simulink model "Intro_PID_Demo"  (R2025b)
settings: Solver=ode45  StartTime=0.0  StopTime=15  MaxStep=0.001  RelTol=1e-6  AbsTol=1e-8
InitFcn:
  | evalin(get_param(bdroot,'ModelWorkspace'),'assert(m>0 && g>0 && a>0 && I>0, ''Physical parameters must be positive.''); assert(F_max>m*g && phi_max>0, ''Limits must allow hover and gimbal movement.''); assert(theta_max>0 && theta_max<=pi/6, ''Use a small positive tilt-command limit.''); assert(numel(X0)==6 && numel(Xref)==6, ''X0 and Xref need six states.''); assert(all(Xref([2 4 5 6])==0), ''Use stationary upright position references.''); assert(all([Kp_x Kd_x Kp_y Kd_y Kp_theta Kd_theta]>0), ''P and D gains must be positive.''); assert(all([Ki_x Ki_y Ki_theta]>=0), ''Integral gains must be nonnegative.'');');
model workspace (MAT data in the model file):
  F_max = 20
  I = 1
  Kd_theta = 1.10091743119
  Kd_x = 1
  Kd_y = 3
  Ki_theta = 0
  Ki_x = 0
  Ki_y = 0
  Kp_theta = 3.66972477064
  Kp_x = 0.25
  Kp_y = 1
  Ts_noise = 0.01
  X0 = [2; 0; 0; 0; 0.03; 0]
  Xref = [3; 0; 30; 0; 0; 0]
  a = 1
  g = 9.81
  m = 1
  phi_max = 0.17
  sigma = [0.03; 0.06; 0.03; 0.06; 0.006; 0.009]
  theta_max = 0.17
libraries: slpidlib x3, simulink x1
settings Model: Creator=cmax0  LastModifiedBy=cmax0

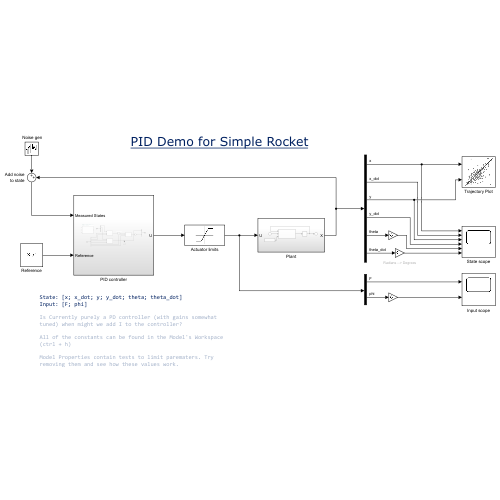
[thumbnail: Simulink's stored preview of the top-level diagram]
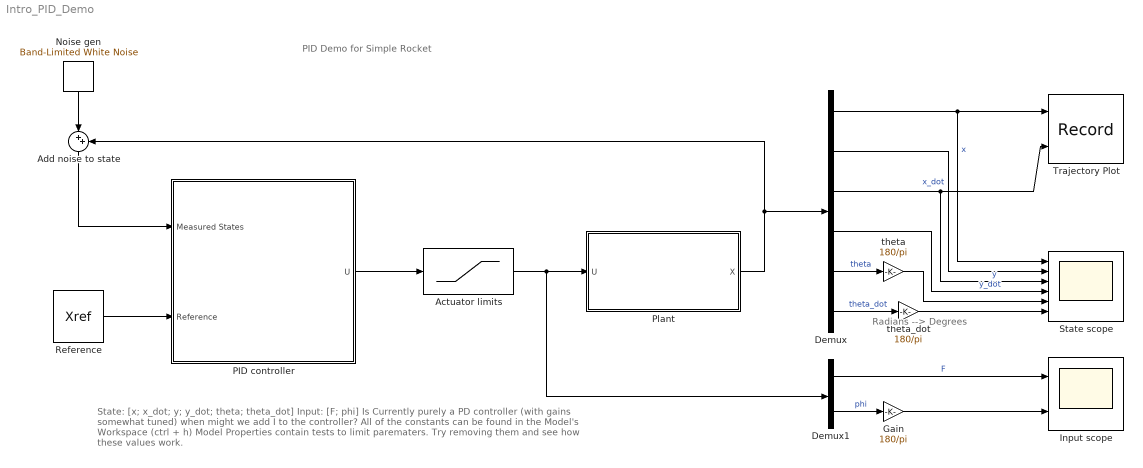
== system Intro_PID_Demo ==
  note: PID Demo for Simple Rocket
  note: State: [x; x_dot; y; y_dot; theta; theta_dot]
      | Input: [F; phi]
      |
      | Is Currently purely a PD controller (with gains somewhat tuned) when might we add I to the controller?
      |
      | All of the constants can be found in the Model's Workspace (ctrl + h)
      |
      | Model Properties contain tests to limit parematers. Try removing them and see how these values work.
  note: Radians --> Degrees
  " Noise gen" : simulink/Sources/Band-Limited White Noise  Cov=sigma.^2 * Ts_noise  Ts=Ts_noise  seed=[11;22;33;44;55;66]
  Actuator limits : Saturate  UpperLimit=[F_max;phi_max]  LowerLimit=[0;-phi_max]
  Add noise to state : Sum  Inputs=|++
  Demux : Demux  Outputs=6
  Demux1 : Demux  Outputs=2
  Gain : Gain  Gain=180/pi
  Input scope : Scope  NumInputPorts=2
      settings: ActiveDisplayYMinimum=-9.207816529611673  ActiveDisplayYMaximum=33.207701324124656
  PID controller : Subsystem
  Plant : Subsystem
  Reference : Constant  Value=Xref
  State scope : Scope  NumInputPorts=6
      settings: ActiveDisplayYMinimum=-27.6164299238122  ActiveDisplayYMaximum=55.714795015888747
  Trajectory Plot : Record  NumPorts=2.0  FileSettingsInternal="{\"entries\":[{\"content\":{\"excelSettings\":{\"content\":{},\"type\":\"Streamout.ExcelSettings\"},\"parquetSettings\":{\"content\":{},\"type\":\"Streamout.ParquetSettings\"}},\"type\":\"Streamout.FileSettingStorage\",\"uuid\":\"\"}],\"packageUris\":[\"http:\\/\\/schema.mathworks.com\\/mf0\\/streamout_blocks\\/R2020a\"],\"version\":\"1.0\"}"  FrameSettings=[0, 0]  Layout=[1 1]  SignalsInternal="{\"entries\":[{\"content\":{\"signals\":[{\"content\":{\"blockPath\":[],\"dimensions\":[1,1],\"domain\":\"\",\"lineColor\":\"#a2142f\",\"plots\":[ 1 ],\"port\":1,\"sid\":[\"\"],\"signalID\":1,\"signalName\":\"x\"},\"type\":\"RecordBlkView.Signal\",\"uuid\":\"\"},{\"content\":{\"blockPath\":[],\"dimensions\":[1,1],\"domain\":\"\",\"lineColor\":\"#139fff\",\"plots\":[ 1 ],\"port\":2,\"sid\":[\"\"],\"signalID\":2,\"signalName\":\"y\"},\"type\":\"RecordBlkView.Signal\",\"uuid\":\"\"}]},\"type\":\"RecordBlkView.InputSignals\",\"uuid\":\"\"}],\"packageUris\":[\"http:\\/\\/schema.mathworks.com\\/mf0\\/streamout_blocks\\/R2020a\"],\"version\":\"1.0\"}"  VisualizationBindings="{\"xyplotplugin\":{\"info\":[{\"series\":[{\"bindingParametersList\":[{\"parameter\":\"X-Axis\",\"signalID\":1,\"signalName\":\"x\"},{\"parameter\":\"Y-Axis\",\"signalID\":2,\"signalName\":\"y\"}],\"seriesID\":0}],\"subplotID\":1}]}}"  CompatibilityTag=XY
  theta : Gain  Gain=180/pi
  theta_dot : Gain  Gain=180/pi
  wires:
  Plant/1(X) -> Add noise to state/2, Demux/1
  Actuator limits/1 -> Plant/1(U), Demux1/1
  " Noise gen"/1 -> Add noise to state/1
  Demux/1 -> Trajectory Plot/1, State scope/1  "x"
  Demux/2 -> State scope/2  "x_dot"
  Demux/3 -> State scope/3, Trajectory Plot/2  "y"
  Demux/5 -> theta/1  "theta"
  Demux/6 -> theta_dot/1  "theta_dot"
  Demux/4 -> State scope/4  "y_dot"
  Demux1/1 -> Input scope/1  "F"
  Demux1/2 -> Gain/1  "phi"
  Reference/1 -> PID controller/2(Reference)
  Add noise to state/1 -> PID controller/1(Measured States)
  PID controller/1(U) -> Actuator limits/1
  Gain/1 -> Input scope/2
  theta_dot/1 -> State scope/6
  theta/1 -> State scope/5

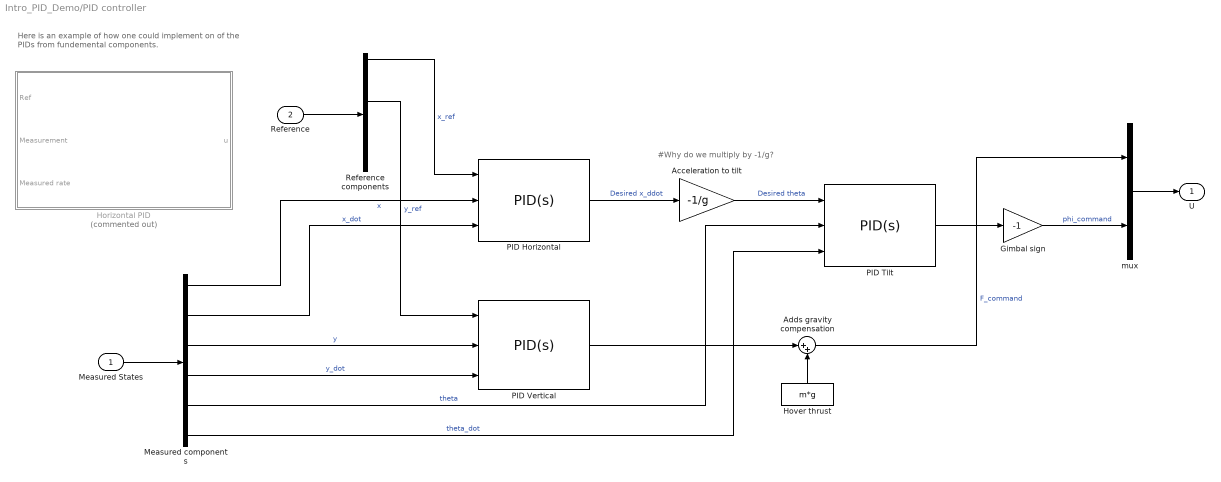
== system Intro_PID_Demo/PID controller ==
  note: Here is an example of how one could implement on of the PIDs from fundemental components.
  note: #Why do we multiply by -1/g?
  Measured States : Inport
  Reference : Inport  Port=2
  Acceleration to tilt : Gain  Gain=-1/g
  Adds gravity compensation : Sum  Inputs=|++
  Gimbal sign : Gain  Gain=-1
  Horizontal PID : Subsystem  Commented=on
  Hover thrust : Constant  Value=m*g
  Measured components : Demux  Outputs=6
  PID Horizontal : slpidlib/PID Controller (2DOF)  Controller=PID  Form=Parallel  TimeDomain=Continuous-time  UseExternalTs=off  SampleTime=-1  IntegratorMethod=Forward Euler  FilterMethod=Forward Euler  ControllerParametersSource=internal  P=Kp_x  I=Ki_x  UseKiTs=off  D=Kd_x  UseExternalDerivativeSource=on  N=100  UseFilter=on  b=1  c=0  TunerSelectOption=Transfer Function Based (PID Tuner App)  InitialConditionSource=internal  InitialConditionForIntegrator=0  InitialConditionForFilter=0  DifferentiatorICPrevScaledInput=0  ExternalReset=none  TrackingMode=off  Kt=1  LimitOutput=on  SatLimitsSource=internal  UpperSaturationLimit=theta_max*g  LowerSaturationLimit=-theta_max*g  LinearizeAsGain=on  AntiWindupMode=clamping  Kb=1  LimitIntegrator=off  UpperIntegratorSaturationLimit=inf  LowerIntegratorSaturationLimit=-inf  POutMin=[]  POutMax=[]  IOutMin=[]  IOutMax=[]  DOutMin=[]  DOutMax=[]  NOutMin=[]  NOutMax=[]  bOutMin=[]  bOutMax=[]  cOutMin=[]  cOutMax=[]  SumOutMin=[]  SumOutMax=[]  SaturationOutMin=[]  SaturationOutMax=[]  PParamMin=[]  PParamMax=[]  IParamMin=[]  IParamMax=[]  DParamMin=[]  DParamMax=[]  NParamMin=[]  NParamMax=[]  bParamMin=[]  bParamMax=[]  cParamMin=[]  cParamMax=[]  KbParamMin=[]  KbParamMax=[]  KtParamMin=[]  KtParamMax=[]  KbOutMin=[]  KbOutMax=[]  KtOutMin=[]  KtOutMax=[]  IntegratorOutMin=[]  IntegratorOutMax=[]  FilterOutMin=[]  FilterOutMax=[]  SumI1OutMin=[]  SumI1OutMax=[]  SumI2OutMin=[]  SumI2OutMax=[]  SumI3OutMin=[]  SumI3OutMax=[]  SumI4OutMin=[]  SumI4OutMax=[]  SumDOutMin=[]  SumDOutMax=[]  Sum1OutMin=[]  Sum1OutMax=[]  Sum2OutMin=[]  Sum2OutMax=[]  Sum3OutMin=[]  Sum3OutMax=[]  DifferentiatorOutMin=[]  DifferentiatorOutMax=[]  FilterDiffOutCoefMin=[]  FilterDiffOutCoefMax=[]  ReciprocalOutMin=[]  ReciprocalOutMax=[]  SumDenOutMin=[]  SumDenOutMax=[]  SumNumOutMin=[]  SumNumOutMax=[]  DivideOutMin=[]  DivideOutMax=[]  UdiffTsProdOutMin=[]  UdiffTsProdOutMax=[]  NTsProdOutMin=[]  NTsProdOutMax=[]  UintegralTsProdOutMin=[]  UintegralTsProdOutMax=[]  UngainTsProdOutMin=[]  UngainTsProdOutMax=[]  ClampingZeroOutDataTypeStr=Inherit: Inherit via back propagation  ClampingZeroOutMin=[]  ClampingZeroOutMax=[]  FilterDenConstantOutDataTypeStr=Inherit: Inherit via back propagation  FilterDenConstantOutMin=[]  FilterDenConstantOutMax=[]  PCopyOutDataTypeStr=Inherit: Inherit via back propagation  PCopyOutMin=[]  PCopyOutMax=[]  NCopyOutDataTypeStr=Inherit: Inherit via back propagation  NCopyOutMin=[]  NCopyOutMax=[]  IntegratorContinuousStateAttributes=''  IntegratorStateMustResolveToSignalObject=off  IntegratorRTWStateStorageClass=Auto  FilterContinuousStateAttributes=''  FilterStateMustResolveToSignalObject=off  FilterRTWStateStorageClass=Auto  ParallelPVariant=InternalParameters  IdealPVariant=Disabled  IVariant=InternalParameters  DVariant=InternalParameters  bVariant=InternalParameters  cVariant=Disabled  IntegratorVariant=Continuous  SatVariant=Enabled  AWVariant=ContClampingParallel  PCopyVariant=Disabled  TRVariant=Disabled  FdbkBlocksVariant=Forward  IdealPFdbkVariant=Disabled  SatFdbkVariant=Disabled  DerivativeFilterVariant=ContFilterOnly  NVariant=InternalParameters  NCopyVariant=Disabled  FilterICVariant=InternalICsFilter  IntegratorICVariant=InternalICs  ExternalResetVariant=Disabled  TRSumVariant=Passthrough  SumFdbkVariant=Disabled  SumVariant=Sum_PID  TsampFilterVariant=InternalTs  TsampNgainVariant=Passthrough  TsampIntegralVariant=Disabled_SignalSpec  ExternalSaturationOutDataTypeStr=Inherit: Same as second input  DerivativeSourceVariant=ExternalYdot  PreIntVariant=InternalPreInt
  PID Tilt : slpidlib/PID Controller (2DOF)  Controller=PID  Form=Parallel  TimeDomain=Continuous-time  UseExternalTs=off  SampleTime=-1  IntegratorMethod=Forward Euler  FilterMethod=Forward Euler  ControllerParametersSource=internal  P=Kp_theta  I=Ki_theta  UseKiTs=off  D=Kd_theta  UseExternalDerivativeSource=on  N=100  UseFilter=on  b=1  c=0  TunerSelectOption=Transfer Function Based (PID Tuner App)  InitialConditionSource=internal  InitialConditionForIntegrator=0  InitialConditionForFilter=0  DifferentiatorICPrevScaledInput=0  ExternalReset=none  TrackingMode=off  Kt=1  LimitOutput=on  SatLimitsSource=internal  UpperSaturationLimit=phi_max  LowerSaturationLimit=-phi_max  LinearizeAsGain=on  AntiWindupMode=clamping  Kb=1  LimitIntegrator=off  UpperIntegratorSaturationLimit=inf  LowerIntegratorSaturationLimit=-inf  POutMin=[]  POutMax=[]  IOutMin=[]  IOutMax=[]  DOutMin=[]  DOutMax=[]  NOutMin=[]  NOutMax=[]  bOutMin=[]  bOutMax=[]  cOutMin=[]  cOutMax=[]  SumOutMin=[]  SumOutMax=[]  SaturationOutMin=[]  SaturationOutMax=[]  PParamMin=[]  PParamMax=[]  IParamMin=[]  IParamMax=[]  DParamMin=[]  DParamMax=[]  NParamMin=[]  NParamMax=[]  bParamMin=[]  bParamMax=[]  cParamMin=[]  cParamMax=[]  KbParamMin=[]  KbParamMax=[]  KtParamMin=[]  KtParamMax=[]  KbOutMin=[]  KbOutMax=[]  KtOutMin=[]  KtOutMax=[]  IntegratorOutMin=[]  IntegratorOutMax=[]  FilterOutMin=[]  FilterOutMax=[]  SumI1OutMin=[]  SumI1OutMax=[]  SumI2OutMin=[]  SumI2OutMax=[]  SumI3OutMin=[]  SumI3OutMax=[]  SumI4OutMin=[]  SumI4OutMax=[]  SumDOutMin=[]  SumDOutMax=[]  Sum1OutMin=[]  Sum1OutMax=[]  Sum2OutMin=[]  Sum2OutMax=[]  Sum3OutMin=[]  Sum3OutMax=[]  DifferentiatorOutMin=[]  DifferentiatorOutMax=[]  FilterDiffOutCoefMin=[]  FilterDiffOutCoefMax=[]  ReciprocalOutMin=[]  ReciprocalOutMax=[]  SumDenOutMin=[]  SumDenOutMax=[]  SumNumOutMin=[]  SumNumOutMax=[]  DivideOutMin=[]  DivideOutMax=[]  UdiffTsProdOutMin=[]  UdiffTsProdOutMax=[]  NTsProdOutMin=[]  NTsProdOutMax=[]  UintegralTsProdOutMin=[]  UintegralTsProdOutMax=[]  UngainTsProdOutMin=[]  UngainTsProdOutMax=[]  ClampingZeroOutDataTypeStr=Inherit: Inherit via back propagation  ClampingZeroOutMin=[]  ClampingZeroOutMax=[]  FilterDenConstantOutDataTypeStr=Inherit: Inherit via back propagation  FilterDenConstantOutMin=[]  FilterDenConstantOutMax=[]  PCopyOutDataTypeStr=Inherit: Inherit via back propagation  PCopyOutMin=[]  PCopyOutMax=[]  NCopyOutDataTypeStr=Inherit: Inherit via back propagation  NCopyOutMin=[]  NCopyOutMax=[]  IntegratorContinuousStateAttributes=''  IntegratorStateMustResolveToSignalObject=off  IntegratorRTWStateStorageClass=Auto  FilterContinuousStateAttributes=''  FilterStateMustResolveToSignalObject=off  FilterRTWStateStorageClass=Auto  ParallelPVariant=InternalParameters  IdealPVariant=Disabled  IVariant=InternalParameters  DVariant=InternalParameters  bVariant=InternalParameters  cVariant=Disabled  IntegratorVariant=Continuous  SatVariant=Enabled  AWVariant=ContClampingParallel  PCopyVariant=Disabled  TRVariant=Disabled  FdbkBlocksVariant=Forward  IdealPFdbkVariant=Disabled  SatFdbkVariant=Disabled  DerivativeFilterVariant=ContFilterOnly  NVariant=InternalParameters  NCopyVariant=Disabled  FilterICVariant=InternalICsFilter  IntegratorICVariant=InternalICs  ExternalResetVariant=Disabled  TRSumVariant=Passthrough  SumFdbkVariant=Disabled  SumVariant=Sum_PID  TsampFilterVariant=InternalTs  TsampNgainVariant=Passthrough  TsampIntegralVariant=Disabled_SignalSpec  ExternalSaturationOutDataTypeStr=Inherit: Same as second input  DerivativeSourceVariant=ExternalYdot  PreIntVariant=InternalPreInt
  PID Vertical : slpidlib/PID Controller (2DOF)  Controller=PID  Form=Parallel  TimeDomain=Continuous-time  UseExternalTs=off  SampleTime=-1  IntegratorMethod=Forward Euler  FilterMethod=Forward Euler  ControllerParametersSource=internal  P=Kp_y  I=Ki_y  UseKiTs=off  D=Kd_y  UseExternalDerivativeSource=on  N=100  UseFilter=on  b=1  c=0  TunerSelectOption=Transfer Function Based (PID Tuner App)  InitialConditionSource=internal  InitialConditionForIntegrator=0  InitialConditionForFilter=0  DifferentiatorICPrevScaledInput=0  ExternalReset=none  TrackingMode=off  Kt=1  LimitOutput=on  SatLimitsSource=internal  UpperSaturationLimit=F_max-m*g  LowerSaturationLimit=-m*g  LinearizeAsGain=on  AntiWindupMode=clamping  Kb=1  LimitIntegrator=off  UpperIntegratorSaturationLimit=inf  LowerIntegratorSaturationLimit=-inf  POutMin=[]  POutMax=[]  IOutMin=[]  IOutMax=[]  DOutMin=[]  DOutMax=[]  NOutMin=[]  NOutMax=[]  bOutMin=[]  bOutMax=[]  cOutMin=[]  cOutMax=[]  SumOutMin=[]  SumOutMax=[]  SaturationOutMin=[]  SaturationOutMax=[]  PParamMin=[]  PParamMax=[]  IParamMin=[]  IParamMax=[]  DParamMin=[]  DParamMax=[]  NParamMin=[]  NParamMax=[]  bParamMin=[]  bParamMax=[]  cParamMin=[]  cParamMax=[]  KbParamMin=[]  KbParamMax=[]  KtParamMin=[]  KtParamMax=[]  KbOutMin=[]  KbOutMax=[]  KtOutMin=[]  KtOutMax=[]  IntegratorOutMin=[]  IntegratorOutMax=[]  FilterOutMin=[]  FilterOutMax=[]  SumI1OutMin=[]  SumI1OutMax=[]  SumI2OutMin=[]  SumI2OutMax=[]  SumI3OutMin=[]  SumI3OutMax=[]  SumI4OutMin=[]  SumI4OutMax=[]  SumDOutMin=[]  SumDOutMax=[]  Sum1OutMin=[]  Sum1OutMax=[]  Sum2OutMin=[]  Sum2OutMax=[]  Sum3OutMin=[]  Sum3OutMax=[]  DifferentiatorOutMin=[]  DifferentiatorOutMax=[]  FilterDiffOutCoefMin=[]  FilterDiffOutCoefMax=[]  ReciprocalOutMin=[]  ReciprocalOutMax=[]  SumDenOutMin=[]  SumDenOutMax=[]  SumNumOutMin=[]  SumNumOutMax=[]  DivideOutMin=[]  DivideOutMax=[]  UdiffTsProdOutMin=[]  UdiffTsProdOutMax=[]  NTsProdOutMin=[]  NTsProdOutMax=[]  UintegralTsProdOutMin=[]  UintegralTsProdOutMax=[]  UngainTsProdOutMin=[]  UngainTsProdOutMax=[]  ClampingZeroOutDataTypeStr=Inherit: Inherit via back propagation  ClampingZeroOutMin=[]  ClampingZeroOutMax=[]  FilterDenConstantOutDataTypeStr=Inherit: Inherit via back propagation  FilterDenConstantOutMin=[]  FilterDenConstantOutMax=[]  PCopyOutDataTypeStr=Inherit: Inherit via back propagation  PCopyOutMin=[]  PCopyOutMax=[]  NCopyOutDataTypeStr=Inherit: Inherit via back propagation  NCopyOutMin=[]  NCopyOutMax=[]  IntegratorContinuousStateAttributes=''  IntegratorStateMustResolveToSignalObject=off  IntegratorRTWStateStorageClass=Auto  FilterContinuousStateAttributes=''  FilterStateMustResolveToSignalObject=off  FilterRTWStateStorageClass=Auto  ParallelPVariant=InternalParameters  IdealPVariant=Disabled  IVariant=InternalParameters  DVariant=InternalParameters  bVariant=InternalParameters  cVariant=Disabled  IntegratorVariant=Continuous  SatVariant=Enabled  AWVariant=ContClampingParallel  PCopyVariant=Disabled  TRVariant=Disabled  FdbkBlocksVariant=Forward  IdealPFdbkVariant=Disabled  SatFdbkVariant=Disabled  DerivativeFilterVariant=ContFilterOnly  NVariant=InternalParameters  NCopyVariant=Disabled  FilterICVariant=InternalICsFilter  IntegratorICVariant=InternalICs  ExternalResetVariant=Disabled  TRSumVariant=Passthrough  SumFdbkVariant=Disabled  SumVariant=Sum_PID  TsampFilterVariant=InternalTs  TsampNgainVariant=Passthrough  TsampIntegralVariant=Disabled_SignalSpec  ExternalSaturationOutDataTypeStr=Inherit: Same as second input  DerivativeSourceVariant=ExternalYdot  PreIntVariant=InternalPreInt
  Reference components : Demux  Outputs=6
  mux : Mux  Inputs=2
  U : Outport
  wires:
  Reference/1 -> Reference components/1
  Measured States/1 -> Measured components/1
  Reference components/1 -> PID Horizontal/1  "x_ref"
  Measured components/1 -> PID Horizontal/2  "x"
  Measured components/2 -> PID Horizontal/3  "x_dot"
  Acceleration to tilt/1 -> PID Tilt/1  "Desired theta"
  Measured components/5 -> PID Tilt/2  "theta"
  Measured components/6 -> PID Tilt/3  "theta_dot"
  PID Tilt/1 -> Gimbal sign/1
  Gimbal sign/1 -> mux/2  "phi_command"
  Reference components/3 -> PID Vertical/1  "y_ref"
  Measured components/3 -> PID Vertical/2  "y"
  Measured components/4 -> PID Vertical/3  "y_dot"
  PID Vertical/1 -> Adds gravity compensation/1
  Adds gravity compensation/1 -> mux/1  "F_command"
  mux/1 -> U/1
  Hover thrust/1 -> Adds gravity compensation/2
  PID Horizontal/1 -> Acceleration to tilt/1  "Desired x_ddot"

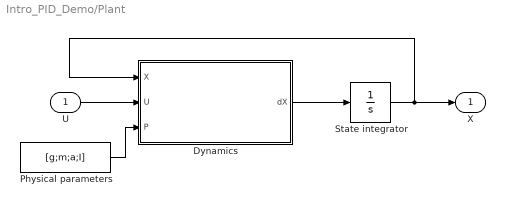
== system Intro_PID_Demo/Plant ==
  U : Inport
  Dynamics : MATLAB Function  TreatAsAtomicUnit=on
  Physical parameters : Constant  Value=[g;m;a;I]
  State integrator : Integrator  InitialCondition=X0
  X : Outport
  wires:
  State integrator/1 -> Dynamics/1(X), X/1
  U/1 -> Dynamics/2(U)
  Physical parameters/1 -> Dynamics/3(P)
  Dynamics/1(dX) -> State integrator/1

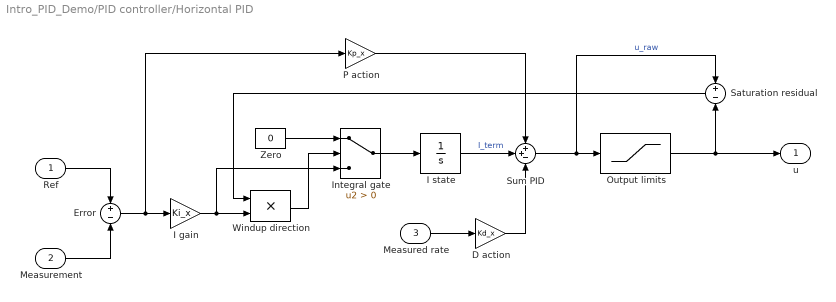
== system Intro_PID_Demo/PID controller/Horizontal PID ==
  Ref : Inport
  Measurement : Inport  Port=2
  Measured rate : Inport  Port=3
  D action : Gain  Gain=Kd_x
  Error : Sum  Inputs=+-
  I gain : Gain  Gain=Ki_x
  I state : Integrator
  Integral gate : Switch  Criteria=u2 > Threshold  SaturateOnIntegerOverflow=off  InputSameDT=off
  Output limits : Saturate  UpperLimit=g*theta_max  LowerLimit=-g*theta_max
  P action : Gain  Gain=Kp_x
  Saturation residual : Sum  Inputs=+-
  Sum PID : Sum  Inputs=++-
  Windup direction : Product  Inputs=**
  Zero : Constant  Value=0
  u : Outport
  wires:
  Error/1 -> P action/1, I gain/1
  Saturation residual/1 -> Windup direction/1
  Measurement/1 -> Error/2
  Ref/1 -> Error/1
  Measured rate/1 -> D action/1
  P action/1 -> Sum PID/1
  Zero/1 -> Integral gate/1
  I gain/1 -> Integral gate/3, Windup direction/2
  Windup direction/1 -> Integral gate/2
  Integral gate/1 -> I state/1
  D action/1 -> Sum PID/3
  I state/1 -> Sum PID/2  "I_term"
  Sum PID/1 -> Saturation residual/1, Output limits/1  "u_raw"
  Output limits/1 -> Saturation residual/2, u/1

== matlab function Intro_PID_Demo/Plant/Dynamics ==
  data: X input size=[6 1]; dX output size=[6 1]; U input size=[2 1]; P input size=[4 1]
function dX = rocketDynamics(X, U, P)

% State: [x; x_dot; y; y_dot; theta; theta_dot]
% Input: [F; phi], Parameters: [g; m; a; I]

g = P(1); m = P(2); a = P(3); I = P(4);
theta = X(5); F = U(1); phi = U(2);

x_ddot = -F/m * sin(theta + phi);
y_ddot = -g + F/m * cos(theta + phi);
theta_ddot = -a * F * sin(phi) / I;

dX = [X(2); x_ddot; X(4); y_ddot; X(6); theta_ddot];
end
